simulink model "analog_current_path"  (R2022b)
settings: Solver=daessc  StartTime=0.0  StopTime=0.2  MaxStep=1e-5  RelTol=1e-3
libraries: fl_lib x59, nesl_utility x5, ee_lib x4
settings Model: Creator=dbagn  LastModifiedBy=ltnbda

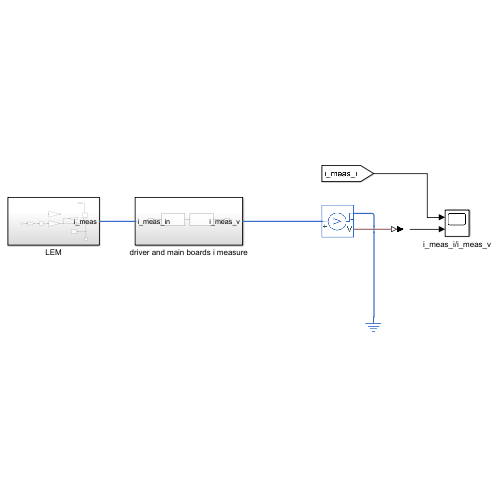
[thumbnail: Simulink's stored preview of the top-level diagram]
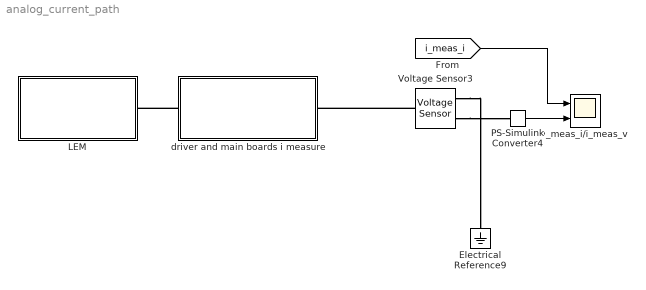
== system analog_current_path ==
  Electrical Reference9 : fl_lib/Electrical/Electrical Elements/Electrical Reference
  LEM : Subsystem
  PS-Simulink Converter4 : nesl_utility/PS-Simulink Converter  PhysicalDomain=network_engine_domain  SubClassName=ps_output  LeftPortType=input  RightPortType=output  PseudoPeriodic=off  Frequencies=[]  VectorFormat=1-D array  Unit=V  AffineConversion=on
  Voltage Sensor3 : fl_lib/Electrical/Electrical Sensors/Voltage Sensor
  driver and main boards i measure : Subsystem
  i_meas_i/i_meas_v : Scope  NumInputPorts=2
  wires:
  PS-Simulink Converter4/1 -> i_meas_i/i_meas_v/2
  [i_meas_i] -> i_meas_i/i_meas_v/1
  connections:
  Voltage Sensor3/RConn2 -- Electrical Reference9/LConn1
  Voltage Sensor3/RConn1 -- PS-Simulink Converter4/LConn1
  driver and main boards i measure/LConn1 -- LEM/LConn1
  Voltage Sensor3/LConn1 -- driver and main boards i measure/RConn1

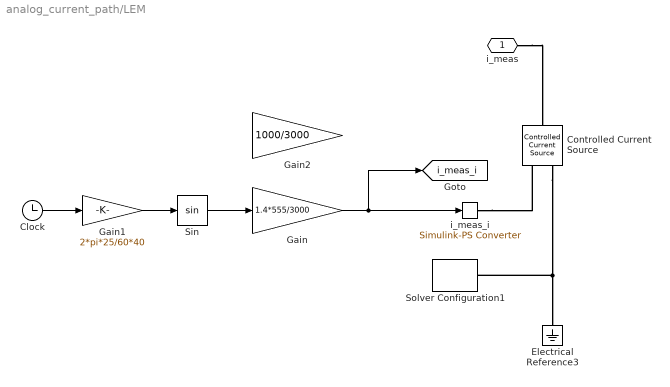
== system analog_current_path/LEM ==
  Clock : Clock
  Controlled Current Source : fl_lib/Electrical/Electrical Sources/Controlled Current Source
  Electrical Reference3 : fl_lib/Electrical/Electrical Elements/Electrical Reference
  Gain : Gain  Gain=1.4*555/3000
  Gain1 : Gain  Gain=2*pi*25/60*40
  Gain2 : Gain  Gain=1000/3000
  Sin : Trigonometry
  Solver Configuration1 : nesl_utility/Solver Configuration  PhysicalDomain=network_engine_domain  SubClassName=solver  LeftPortType=input  RightPortType=generic  Tones=[]  Harmonics=[]  SimulateNoise=off  Profile=off  UseLocalSampling=off  EnableSwitchedLinearOptims=on  FrequencyDomain=off  UseCCode=off  RelTol=0.001  AbsTol=1e-06  MinStep=1e-09  ToWorkspace=off  RevertToSquareIcSolve=off  NumHomotopyIterations=100  PhasorMode=off  PhasorModeNumHarmonics=1  ConsistencySolver=NEWTON_FTOL  IndexReductionMethod=DerivativeReplacement  DoDC=off  ResidualTolerance=1e-09  ConsistencyTolSource=GLOBAL  ConsistencyAbsTol=0.001  ConsistencyRelTol=0.001  ConsistencyTolFactor=0.001  UseLocalSolver=off  LocalSolverChoice=NE_BACKWARD_EULER_ADVANCER  ResolveIndetEquations=on  FunctionEvalNumThread=1  LocalSolverSampleTime=0.001  DoFixedCost=off  MaxNonlinIter=3  MaxModeIter=2  ComputeImpulses=off  ImpulseIterations=2  LinearAlgebra=auto  LinearAlgebraNumThread=0  EquationFormulation=NE_TIME_EF  DelaysMemoryBudget=1024  AutomaticFiltering=on  FilteringTimeConstant=0.001  PartitionStorageMethod=AS_NEEDED  PartitionMemoryBudget=1024  PartitionMethod=ROBUST
  i_meas_i : nesl_utility/Simulink-PS Converter  PhysicalDomain=network_engine_domain  SubClassName=ps_input  LeftPortType=input  RightPortType=output  PseudoPeriodic=off  Frequencies=[]  NoiseDistribution=none  NoiseParameters=[]  Unit=A  AffineConversion=on  FilteringAndDerivatives=provide  SimscapeFilterOrder=1  InputFilterTimeConstant=0.001  UdotUserProvided=0
  i_meas : PMIOPort  Side=Left
  tag scope: i_meas_i=global
  wires:
  Sin/1 -> Gain/1
  Gain/1 -> [i_meas_i], i_meas_i/1
  Gain1/1 -> Sin/1
  Clock/1 -> Gain1/1
  connections:
  i_meas/RConn1 -- Controlled Current Source/LConn1
  i_meas_i/RConn1 -- Controlled Current Source/RConn1
  Controlled Current Source/RConn2 -- Electrical Reference3/LConn1 -- Solver Configuration1/RConn1

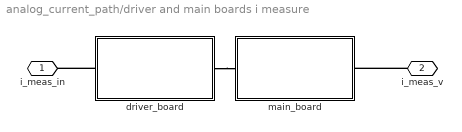
== system analog_current_path/driver and main boards i measure ==
  driver_board : Subsystem
  main_board : Subsystem
  i_meas_in : PMIOPort  Side=Left
  i_meas_v : PMIOPort  Port=2  Side=Right
  connections:
  driver_board/RConn1 -- main_board/LConn1
  i_meas_v/RConn1 -- main_board/RConn1
  driver_board/LConn1 -- i_meas_in/RConn1

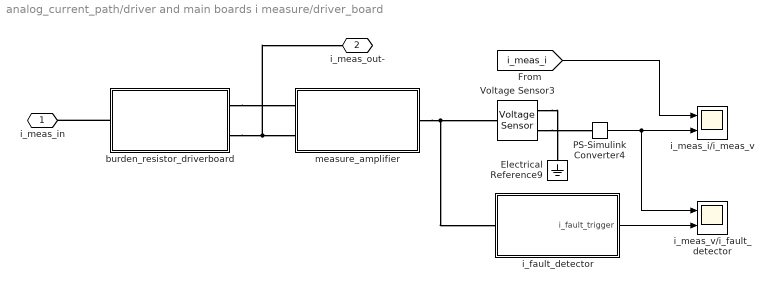
== system analog_current_path/driver and main boards i measure/driver_board ==
  Electrical Reference9 : fl_lib/Electrical/Electrical Elements/Electrical Reference
  PS-Simulink Converter4 : nesl_utility/PS-Simulink Converter  PhysicalDomain=network_engine_domain  SubClassName=ps_output  LeftPortType=input  RightPortType=output  PseudoPeriodic=off  Frequencies=[]  VectorFormat=1-D array  Unit=V  AffineConversion=on
  Voltage Sensor3 : fl_lib/Electrical/Electrical Sensors/Voltage Sensor
  burden_resistor_driverboard : Subsystem
  i_fault_detector : Subsystem
  i_meas_i/i_meas_v : Scope  NumInputPorts=2
  i_meas_v/i_fault_detector : Scope  NumInputPorts=2
  measure_amplifier : Subsystem
  i_meas_in : PMIOPort  Side=Left
  i_meas_out- : PMIOPort  Port=2  Side=Right
  wires:
  PS-Simulink Converter4/1 -> i_meas_v/i_fault_detector/1, i_meas_i/i_meas_v/2
  [i_meas_i] -> i_meas_i/i_meas_v/1
  i_fault_detector/1(i_fault_trigger) -> i_meas_v/i_fault_detector/2
  connections:
  burden_resistor_driverboard/LConn1 -- i_meas_in/RConn1
  burden_resistor_driverboard/RConn2 -- i_meas_out-/RConn1 -- measure_amplifier/LConn2
  burden_resistor_driverboard/RConn1 -- measure_amplifier/LConn1
  Voltage Sensor3/RConn1 -- PS-Simulink Converter4/LConn1
  measure_amplifier/RConn1 -- i_fault_detector/LConn1 -- Voltage Sensor3/LConn1
  Voltage Sensor3/RConn2 -- Electrical Reference9/LConn1

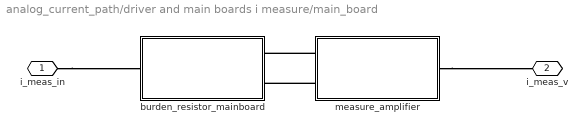
== system analog_current_path/driver and main boards i measure/main_board ==
  burden_resistor_mainboard : Subsystem
  measure_amplifier : Subsystem
  i_meas_in : PMIOPort  Side=Left
  i_meas_v : PMIOPort  Port=2  Side=Right
  connections:
  measure_amplifier/LConn1 -- burden_resistor_mainboard/RConn1
  measure_amplifier/RConn1 -- i_meas_v/RConn1
  i_meas_in/RConn1 -- burden_resistor_mainboard/LConn1
  measure_amplifier/LConn2 -- burden_resistor_mainboard/RConn2

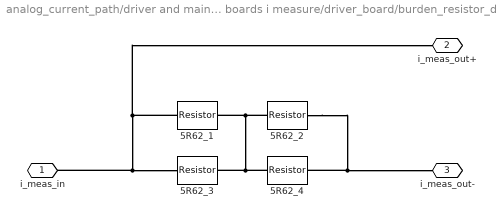
== system analog_current_path/driver and main boards i measure/driver_board/burden_resistor_driverboard ==
  5R62_{1..4} (4 alike) : fl_lib/Electrical/Electrical Elements/Resistor  R=5.62 Ohm  i_specify=off  i_priority=None  i=0 A  i_nominal_specify=off  i_nominal_unit=A  i_nominal_value=1  v_specify=off  v_priority=None  v=0 V  v_nominal_specify=off  v_nominal_unit=V  v_nominal_value=1
  i_meas_in : PMIOPort  Side=Left
  i_meas_out+ : PMIOPort  Port=2  Side=Right
  i_meas_out- : PMIOPort  Port=3  Side=Right
  connections:
  5R62_2/LConn1 -- 5R62_3/RConn1 -- 5R62_4/LConn1 -- 5R62_1/RConn1
  5R62_1/LConn1 -- i_meas_in/RConn1 -- 5R62_3/LConn1 -- i_meas_out+/RConn1
  5R62_2/RConn1 -- i_meas_out-/RConn1 -- 5R62_4/RConn1

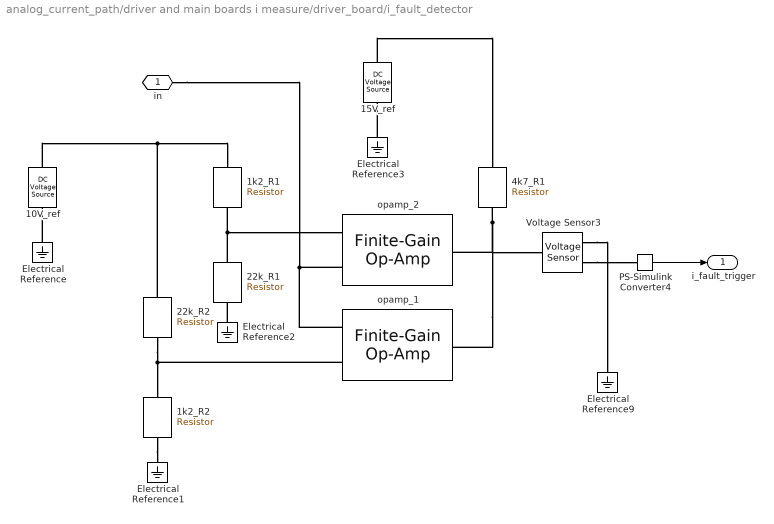
== system analog_current_path/driver and main boards i measure/driver_board/i_fault_detector ==
  10V_ref : fl_lib/Electrical/Electrical Sources/DC Voltage Source  v0=10 V
  15V_ref : fl_lib/Electrical/Electrical Sources/DC Voltage Source  v0=10 V
  1k2_R1 : fl_lib/Electrical/Electrical Elements/Resistor  R=1200 Ohm  i_specify=off  i_priority=None  i=0 A  i_nominal_specify=off  i_nominal_unit=A  i_nominal_value=1  v_specify=off  v_priority=None  v=0 V  v_nominal_specify=off  v_nominal_unit=V  v_nominal_value=1
  1k2_R2 : fl_lib/Electrical/Electrical Elements/Resistor  R=1200 Ohm  i_specify=off  i_priority=None  i=0 A  i_nominal_specify=off  i_nominal_unit=A  i_nominal_value=1  v_specify=off  v_priority=None  v=0 V  v_nominal_specify=off  v_nominal_unit=V  v_nominal_value=1
  22k_R1 : fl_lib/Electrical/Electrical Elements/Resistor  R=22e3 Ohm  i_specify=off  i_priority=None  i=0 A  i_nominal_specify=off  i_nominal_unit=A  i_nominal_value=1  v_specify=off  v_priority=None  v=0 V  v_nominal_specify=off  v_nominal_unit=V  v_nominal_value=1
  22k_R2 : fl_lib/Electrical/Electrical Elements/Resistor  R=22e3 Ohm  i_specify=off  i_priority=None  i=0 A  i_nominal_specify=off  i_nominal_unit=A  i_nominal_value=1  v_specify=off  v_priority=None  v=0 V  v_nominal_specify=off  v_nominal_unit=V  v_nominal_value=1
  4k7_R1 : fl_lib/Electrical/Electrical Elements/Resistor  R=4700 Ohm  i_specify=off  i_priority=None  i=0 A  i_nominal_specify=off  i_nominal_unit=A  i_nominal_value=1  v_specify=off  v_priority=None  v=0 V  v_nominal_specify=off  v_nominal_unit=V  v_nominal_value=1
  Electrical Reference{,1..3,9} (5 alike) : fl_lib/Electrical/Electrical Elements/Electrical Reference
  PS-Simulink Converter4 : nesl_utility/PS-Simulink Converter  PhysicalDomain=network_engine_domain  SubClassName=ps_output  LeftPortType=input  RightPortType=output  PseudoPeriodic=off  Frequencies=[]  VectorFormat=1-D array  Unit=V  AffineConversion=on
  Voltage Sensor3 : fl_lib/Electrical/Electrical Sensors/Voltage Sensor
  opamp_1 : ee_lib/Integrated Circuits/Finite-Gain Op-Amp  A=5e6  Rin=1e6 Ohm  Rout=100 Ohm  Vmin=-12 V  Vmax=+12 V  noise_mode=0  v_noise=30e-9 V/Hz^0.50000  noise_prm=1  i_noise=0.5e-12 A/Hz^0.50000  ip_noise=0.5e-12 A/Hz^0.50000  in_noise=0.5e-12 A/Hz^0.50000  sample_time=1e-3 s  repeatability=1  auto_seed_v=153380492  auto_seed_ip=3646982598  auto_seed_in=4011470453  user_seed_v=0  user_seed_ip=0  user_seed_in=0
      settings: InternalSimscapePortConfiguration="{\"Bottom\":[],\"Left\":[{\"id\":\"p\",\"label\":\"+\",\"type\":\"foundation.electrical.electrical\"},{\"id\":\"n\",\"label\":\"-\",\"type\":\"foundation.electrical.electrical\"}],\"Right\":[{\"id\":\"out\",\"label\":\"\",\"type\":\"foundation.electrical.electrical\"}],\"Top\":[]}"
  opamp_2 : ee_lib/Integrated Circuits/Finite-Gain Op-Amp  A=5e6  Rin=1e6 Ohm  Rout=100 Ohm  Vmin=-12 V  Vmax=+12 V  noise_mode=0  v_noise=30e-9 V/Hz^0.50000  noise_prm=1  i_noise=0.5e-12 A/Hz^0.50000  ip_noise=0.5e-12 A/Hz^0.50000  in_noise=0.5e-12 A/Hz^0.50000  sample_time=1e-3 s  repeatability=1  auto_seed_v=2915145293  auto_seed_ip=3254469079  auto_seed_in=3191729647  user_seed_v=0  user_seed_ip=0  user_seed_in=0
      settings: InternalSimscapePortConfiguration="{\"Bottom\":[],\"Left\":[{\"id\":\"p\",\"label\":\"+\",\"type\":\"foundation.electrical.electrical\"},{\"id\":\"n\",\"label\":\"-\",\"type\":\"foundation.electrical.electrical\"}],\"Right\":[{\"id\":\"out\",\"label\":\"\",\"type\":\"foundation.electrical.electrical\"}],\"Top\":[]}"
  in : PMIOPort  Side=Left
  i_fault_trigger : Outport
  wires:
  PS-Simulink Converter4/1 -> i_fault_trigger/1
  connections:
  Electrical Reference/LConn1 -- 10V_ref/RConn1
  in/RConn1 -- opamp_2/LConn2 -- opamp_1/LConn1
  10V_ref/LConn1 -- 22k_R2/LConn1 -- 1k2_R1/LConn1
  22k_R1/LConn1 -- opamp_2/LConn1 -- 1k2_R1/RConn1
  Electrical Reference2/LConn1 -- 22k_R1/RConn1
  1k2_R2/RConn1 -- Electrical Reference1/LConn1
  22k_R2/RConn1 -- 1k2_R2/LConn1 -- opamp_1/LConn2
  Electrical Reference3/LConn1 -- 15V_ref/RConn1
  15V_ref/LConn1 -- 4k7_R1/LConn1
  4k7_R1/RConn1 -- Voltage Sensor3/LConn1 -- opamp_1/RConn1 -- opamp_2/RConn1
  Voltage Sensor3/RConn1 -- PS-Simulink Converter4/LConn1
  Voltage Sensor3/RConn2 -- Electrical Reference9/LConn1

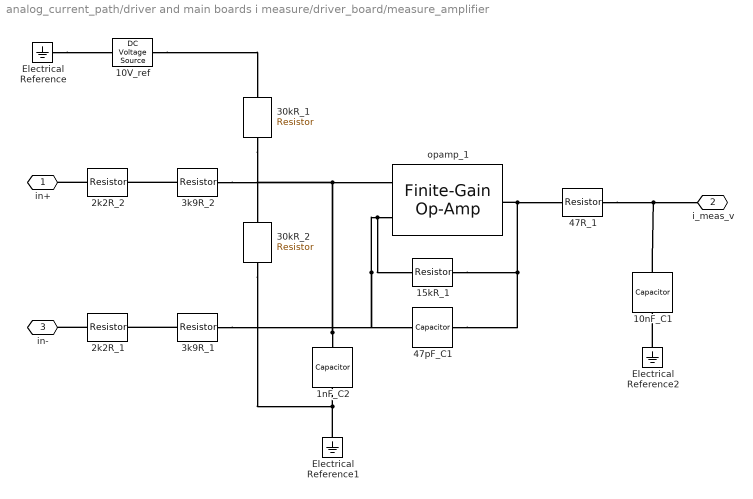
== system analog_current_path/driver and main boards i measure/driver_board/measure_amplifier ==
  10V_ref : fl_lib/Electrical/Electrical Sources/DC Voltage Source  v0=10 V
  10nF_C1 : fl_lib/Electrical/Electrical Elements/Capacitor  c=10e-9 F  r=1e-6 Ohm  g=0 1/Ohm  i_specify=off  i_priority=None  i=0 A  i_nominal_specify=off  i_nominal_unit=A  i_nominal_value=1  v_specify=off  v_priority=None  v=0 V  v_nominal_specify=off  v_nominal_unit=V  v_nominal_value=1  vc_specify=off  vc_priority=High  vc=0 V  vc_nominal_specify=off  vc_nominal_unit=V  vc_nominal_value=1
  15kR_1 : fl_lib/Electrical/Electrical Elements/Resistor  R=15e3 Ohm  i_specify=off  i_priority=None  i=0 A  i_nominal_specify=off  i_nominal_unit=A  i_nominal_value=1  v_specify=off  v_priority=None  v=0 V  v_nominal_specify=off  v_nominal_unit=V  v_nominal_value=1
  1nF_C2 : fl_lib/Electrical/Electrical Elements/Capacitor  c=1e-9 F  r=1e-6 Ohm  g=0 1/Ohm  i_specify=off  i_priority=None  i=0 A  i_nominal_specify=off  i_nominal_unit=A  i_nominal_value=1  v_specify=off  v_priority=None  v=0 V  v_nominal_specify=off  v_nominal_unit=V  v_nominal_value=1  vc_specify=off  vc_priority=High  vc=0 V  vc_nominal_specify=off  vc_nominal_unit=V  vc_nominal_value=1
  2k2R_1 : fl_lib/Electrical/Electrical Elements/Resistor  R=2200 Ohm  i_specify=off  i_priority=None  i=0 A  i_nominal_specify=off  i_nominal_unit=A  i_nominal_value=1  v_specify=off  v_priority=None  v=0 V  v_nominal_specify=off  v_nominal_unit=V  v_nominal_value=1
  2k2R_2 : fl_lib/Electrical/Electrical Elements/Resistor  R=2200 Ohm  i_specify=off  i_priority=None  i=0 A  i_nominal_specify=off  i_nominal_unit=A  i_nominal_value=1  v_specify=off  v_priority=None  v=0 V  v_nominal_specify=off  v_nominal_unit=V  v_nominal_value=1
  30kR_1 : fl_lib/Electrical/Electrical Elements/Resistor  R=30e3 Ohm  i_specify=off  i_priority=None  i=0 A  i_nominal_specify=off  i_nominal_unit=A  i_nominal_value=1  v_specify=off  v_priority=None  v=0 V  v_nominal_specify=off  v_nominal_unit=V  v_nominal_value=1
  30kR_2 : fl_lib/Electrical/Electrical Elements/Resistor  R=30e3 Ohm  i_specify=off  i_priority=None  i=0 A  i_nominal_specify=off  i_nominal_unit=A  i_nominal_value=1  v_specify=off  v_priority=None  v=0 V  v_nominal_specify=off  v_nominal_unit=V  v_nominal_value=1
  3k9R_1 : fl_lib/Electrical/Electrical Elements/Resistor  R=3900 Ohm  i_specify=off  i_priority=None  i=0 A  i_nominal_specify=off  i_nominal_unit=A  i_nominal_value=1  v_specify=off  v_priority=None  v=0 V  v_nominal_specify=off  v_nominal_unit=V  v_nominal_value=1
  3k9R_2 : fl_lib/Electrical/Electrical Elements/Resistor  R=3900 Ohm  i_specify=off  i_priority=None  i=0 A  i_nominal_specify=off  i_nominal_unit=A  i_nominal_value=1  v_specify=off  v_priority=None  v=0 V  v_nominal_specify=off  v_nominal_unit=V  v_nominal_value=1
  47R_1 : fl_lib/Electrical/Electrical Elements/Resistor  R=47 Ohm  i_specify=off  i_priority=None  i=0 A  i_nominal_specify=off  i_nominal_unit=A  i_nominal_value=1  v_specify=off  v_priority=None  v=0 V  v_nominal_specify=off  v_nominal_unit=V  v_nominal_value=1
  47pF_C1 : fl_lib/Electrical/Electrical Elements/Capacitor  c=47e-12 F  r=1e-6 Ohm  g=0 1/Ohm  i_specify=off  i_priority=None  i=0 A  i_nominal_specify=off  i_nominal_unit=A  i_nominal_value=1  v_specify=off  v_priority=None  v=0 V  v_nominal_specify=off  v_nominal_unit=V  v_nominal_value=1  vc_specify=off  vc_priority=High  vc=0 V  vc_nominal_specify=off  vc_nominal_unit=V  vc_nominal_value=1
  Electrical Reference : fl_lib/Electrical/Electrical Elements/Electrical Reference
  Electrical Reference1 : fl_lib/Electrical/Electrical Elements/Electrical Reference
  Electrical Reference2 : fl_lib/Electrical/Electrical Elements/Electrical Reference
  opamp_1 : ee_lib/Integrated Circuits/Finite-Gain Op-Amp  A=5e6  Rin=1e6 Ohm  Rout=100 Ohm  Vmin=-12 V  Vmax=+12 V  noise_mode=0  v_noise=30e-9 V/Hz^0.50000  noise_prm=1  i_noise=0.5e-12 A/Hz^0.50000  ip_noise=0.5e-12 A/Hz^0.50000  in_noise=0.5e-12 A/Hz^0.50000  sample_time=1e-3 s  repeatability=1  auto_seed_v=4111000739  auto_seed_ip=2084672538  auto_seed_in=3437178441  user_seed_v=0  user_seed_ip=0  user_seed_in=0
      settings: InternalSimscapePortConfiguration="{\"Bottom\":[],\"Left\":[{\"id\":\"p\",\"label\":\"+\",\"type\":\"foundation.electrical.electrical\"},{\"id\":\"n\",\"label\":\"-\",\"type\":\"foundation.electrical.electrical\"}],\"Right\":[{\"id\":\"out\",\"label\":\"\",\"type\":\"foundation.electrical.electrical\"}],\"Top\":[]}"
  in+ : PMIOPort  Side=Left
  i_meas_v : PMIOPort  Port=2  Side=Right
  in- : PMIOPort  Port=3  Side=Left
  connections:
  opamp_1/LConn2 -- 15kR_1/LConn1 -- 3k9R_1/RConn1 -- 47pF_C1/LConn1
  3k9R_1/LConn1 -- 2k2R_1/RConn1
  1nF_C2/LConn1 -- opamp_1/LConn1 -- 30kR_2/LConn1 -- 3k9R_2/RConn1 -- 30kR_1/RConn1
  2k2R_2/LConn1 -- in+/RConn1
  2k2R_1/LConn1 -- in-/RConn1
  47pF_C1/RConn1 -- 15kR_1/RConn1 -- opamp_1/RConn1 -- 47R_1/LConn1
  Electrical Reference/LConn1 -- 10V_ref/RConn1
  Electrical Reference1/LConn1 -- 30kR_2/RConn1 -- 1nF_C2/RConn1
  10V_ref/LConn1 -- 30kR_1/LConn1
  3k9R_2/LConn1 -- 2k2R_2/RConn1
  Electrical Reference2/LConn1 -- 10nF_C1/RConn1
  47R_1/RConn1 -- 10nF_C1/LConn1 -- i_meas_v/RConn1

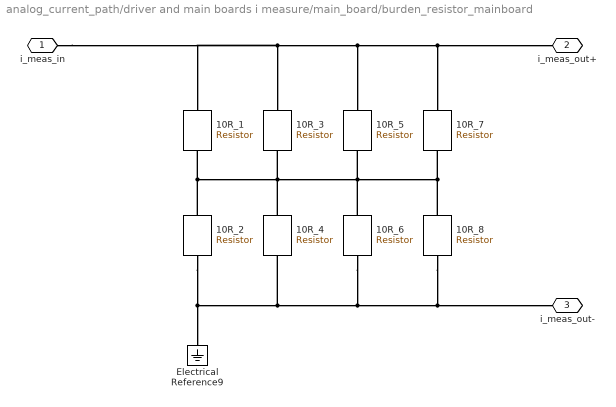
== system analog_current_path/driver and main boards i measure/main_board/burden_resistor_mainboard ==
  10R_{1..8} (8 alike) : fl_lib/Electrical/Electrical Elements/Resistor  R=10 Ohm  i_specify=off  i_priority=None  i=0 A  i_nominal_specify=off  i_nominal_unit=A  i_nominal_value=1  v_specify=off  v_priority=None  v=0 V  v_nominal_specify=off  v_nominal_unit=V  v_nominal_value=1
  Electrical Reference9 : fl_lib/Electrical/Electrical Elements/Electrical Reference
  i_meas_in : PMIOPort  Side=Left
  i_meas_out+ : PMIOPort  Port=2  Side=Right
  i_meas_out- : PMIOPort  Port=3  Side=Right
  connections:
  10R_2/RConn1 -- Electrical Reference9/LConn1 -- 10R_4/RConn1 -- 10R_6/RConn1 -- i_meas_out-/RConn1 -- 10R_8/RConn1
  10R_1/LConn1 -- i_meas_in/RConn1 -- 10R_3/LConn1 -- 10R_5/LConn1 -- i_meas_out+/RConn1 -- 10R_7/LConn1
  10R_2/LConn1 -- 10R_1/RConn1 -- 10R_3/RConn1 -- 10R_4/LConn1 -- 10R_8/LConn1 -- 10R_7/RConn1 -- 10R_5/RConn1 -- 10R_6/LConn1

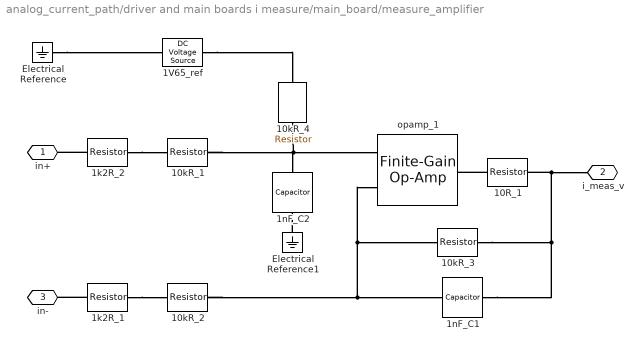
== system analog_current_path/driver and main boards i measure/main_board/measure_amplifier ==
  10R_1 : fl_lib/Electrical/Electrical Elements/Resistor  R=10 Ohm  i_specify=off  i_priority=None  i=0 A  i_nominal_specify=off  i_nominal_unit=A  i_nominal_value=1  v_specify=off  v_priority=None  v=0 V  v_nominal_specify=off  v_nominal_unit=V  v_nominal_value=1
  10kR_{1..4} (4 alike) : fl_lib/Electrical/Electrical Elements/Resistor  R=10e3 Ohm  i_specify=off  i_priority=None  i=0 A  i_nominal_specify=off  i_nominal_unit=A  i_nominal_value=1  v_specify=off  v_priority=None  v=0 V  v_nominal_specify=off  v_nominal_unit=V  v_nominal_value=1
  1V65_ref : fl_lib/Electrical/Electrical Sources/DC Voltage Source  v0=1.65 V
  1k2R_1 : fl_lib/Electrical/Electrical Elements/Resistor  R=1200 Ohm  i_specify=off  i_priority=None  i=0 A  i_nominal_specify=off  i_nominal_unit=A  i_nominal_value=1  v_specify=off  v_priority=None  v=0 V  v_nominal_specify=off  v_nominal_unit=V  v_nominal_value=1
  1k2R_2 : fl_lib/Electrical/Electrical Elements/Resistor  R=1200 Ohm  i_specify=off  i_priority=None  i=0 A  i_nominal_specify=off  i_nominal_unit=A  i_nominal_value=1  v_specify=off  v_priority=None  v=0 V  v_nominal_specify=off  v_nominal_unit=V  v_nominal_value=1
  1nF_C1 : fl_lib/Electrical/Electrical Elements/Capacitor  c=1e-9 F  r=1e-6 Ohm  g=0 1/Ohm  i_specify=off  i_priority=None  i=0 A  i_nominal_specify=off  i_nominal_unit=A  i_nominal_value=1  v_specify=off  v_priority=None  v=0 V  v_nominal_specify=off  v_nominal_unit=V  v_nominal_value=1  vc_specify=off  vc_priority=High  vc=0 V  vc_nominal_specify=off  vc_nominal_unit=V  vc_nominal_value=1
  1nF_C2 : fl_lib/Electrical/Electrical Elements/Capacitor  c=1e-9 F  r=1e-6 Ohm  g=0 1/Ohm  i_specify=off  i_priority=None  i=0 A  i_nominal_specify=off  i_nominal_unit=A  i_nominal_value=1  v_specify=off  v_priority=None  v=0 V  v_nominal_specify=off  v_nominal_unit=V  v_nominal_value=1  vc_specify=off  vc_priority=High  vc=0 V  vc_nominal_specify=off  vc_nominal_unit=V  vc_nominal_value=1
  Electrical Reference : fl_lib/Electrical/Electrical Elements/Electrical Reference
  Electrical Reference1 : fl_lib/Electrical/Electrical Elements/Electrical Reference
  opamp_1 : ee_lib/Integrated Circuits/Finite-Gain Op-Amp  A=5e6  Rin=1e6 Ohm  Rout=100 Ohm  Vmin=-12 V  Vmax=+12 V  noise_mode=0  v_noise=30e-9 V/Hz^0.50000  noise_prm=1  i_noise=0.5e-12 A/Hz^0.50000  ip_noise=0.5e-12 A/Hz^0.50000  in_noise=0.5e-12 A/Hz^0.50000  sample_time=1e-3 s  repeatability=1  auto_seed_v=4144164703  auto_seed_ip=676943032  auto_seed_in=4168664255  user_seed_v=0  user_seed_ip=0  user_seed_in=0
      settings: InternalSimscapePortConfiguration="{\"Bottom\":[],\"Left\":[{\"id\":\"p\",\"label\":\"+\",\"type\":\"foundation.electrical.electrical\"},{\"id\":\"n\",\"label\":\"-\",\"type\":\"foundation.electrical.electrical\"}],\"Right\":[{\"id\":\"out\",\"label\":\"\",\"type\":\"foundation.electrical.electrical\"}],\"Top\":[]}"
  in+ : PMIOPort  Side=Left
  i_meas_v : PMIOPort  Port=2  Side=Right
  in- : PMIOPort  Port=3  Side=Left
  connections:
  10kR_2/RConn1 -- opamp_1/LConn2 -- 10kR_3/LConn1 -- 1nF_C1/LConn1
  1k2R_2/RConn1 -- 10kR_1/LConn1
  1k2R_1/RConn1 -- 10kR_2/LConn1
  10kR_1/RConn1 -- 10kR_4/RConn1 -- 1nF_C2/LConn1 -- opamp_1/LConn1
  10kR_3/RConn1 -- 1nF_C1/RConn1 -- i_meas_v/RConn1 -- 10R_1/RConn1
  1k2R_2/LConn1 -- in+/RConn1
  1k2R_1/LConn1 -- in-/RConn1
  10R_1/LConn1 -- opamp_1/RConn1
  Electrical Reference/LConn1 -- 1V65_ref/RConn1
  Electrical Reference1/LConn1 -- 1nF_C2/RConn1
  1V65_ref/LConn1 -- 10kR_4/LConn1
